simulink model "WarehousePhase2Sim"  (R2024b)
settings: Solver=ode4  StartTime=0.0  StopTime=inf  FixedStep=0.02  RelTol=1e-3
StopFcn:
  | try, fleetVisionStep('close'); catch, end; try, phase2('stopped'); catch, end
model workspace (MAT data in the model file):
  HomePose1 = [-20 7.3 0]
  Zero = 0
  gen3 : robotics.RigidBodyTree (value not decoded)
  qStow = [0; 0; 0.261799387799; 3.14159265359; -2.26892802759; 0; 0.959931088597; 1.57079632679]
undefined symbols (not defined in the file or in its folder): Actor, setupFleetScene, Sim3dSensor, World
libraries: sim3dlib x113, sim3dcameralib x2, robotmobilelib x1, robotsim3dlib x1
(part 2 of 2)

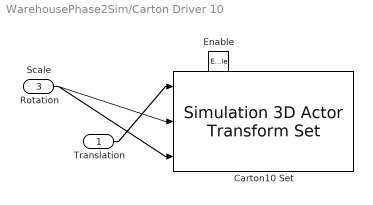
== system WarehousePhase2Sim/Carton Driver 10 ==
  Translation : Inport
  Rotation : Inport  Port=2
  Scale : Inport  Port=3
  Enable : EnablePort
  Carton10 Set : sim3dlib/Simulation 3D Actor Transform Set  Priority=1  ActorTag=Carton10  NumberOfParts=1  CustNumOfParts=3  Translation=[0 0 0]  Rotation=[0 0 0]  Scale=[1 1 1]  Ts=-1  aMode=aMode
  wires:
  Translation/1 -> Carton10 Set/1
  Rotation/1 -> Carton10 Set/2
  Scale/1 -> Carton10 Set/3

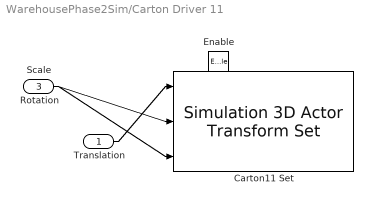
== system WarehousePhase2Sim/Carton Driver 11 ==
  Translation : Inport
  Rotation : Inport  Port=2
  Scale : Inport  Port=3
  Enable : EnablePort
  Carton11 Set : sim3dlib/Simulation 3D Actor Transform Set  Priority=1  ActorTag=Carton11  NumberOfParts=1  CustNumOfParts=3  Translation=[0 0 0]  Rotation=[0 0 0]  Scale=[1 1 1]  Ts=-1  aMode=aMode
  wires:
  Translation/1 -> Carton11 Set/1
  Rotation/1 -> Carton11 Set/2
  Scale/1 -> Carton11 Set/3

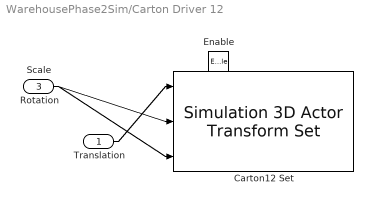
== system WarehousePhase2Sim/Carton Driver 12 ==
  Translation : Inport
  Rotation : Inport  Port=2
  Scale : Inport  Port=3
  Enable : EnablePort
  Carton12 Set : sim3dlib/Simulation 3D Actor Transform Set  Priority=1  ActorTag=Carton12  NumberOfParts=1  CustNumOfParts=3  Translation=[0 0 0]  Rotation=[0 0 0]  Scale=[1 1 1]  Ts=-1  aMode=aMode
  wires:
  Translation/1 -> Carton12 Set/1
  Rotation/1 -> Carton12 Set/2
  Scale/1 -> Carton12 Set/3

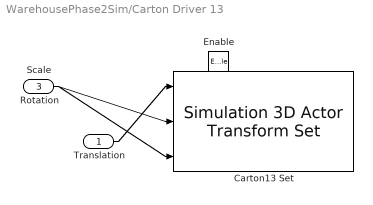
== system WarehousePhase2Sim/Carton Driver 13 ==
  Translation : Inport
  Rotation : Inport  Port=2
  Scale : Inport  Port=3
  Enable : EnablePort
  Carton13 Set : sim3dlib/Simulation 3D Actor Transform Set  Priority=1  ActorTag=Carton13  NumberOfParts=1  CustNumOfParts=3  Translation=[0 0 0]  Rotation=[0 0 0]  Scale=[1 1 1]  Ts=-1  aMode=aMode
  wires:
  Translation/1 -> Carton13 Set/1
  Rotation/1 -> Carton13 Set/2
  Scale/1 -> Carton13 Set/3

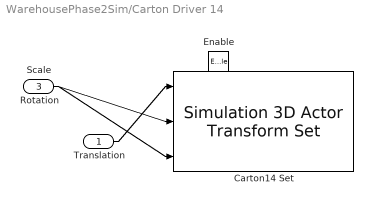
== system WarehousePhase2Sim/Carton Driver 14 ==
  Translation : Inport
  Rotation : Inport  Port=2
  Scale : Inport  Port=3
  Enable : EnablePort
  Carton14 Set : sim3dlib/Simulation 3D Actor Transform Set  Priority=1  ActorTag=Carton14  NumberOfParts=1  CustNumOfParts=3  Translation=[0 0 0]  Rotation=[0 0 0]  Scale=[1 1 1]  Ts=-1  aMode=aMode
  wires:
  Translation/1 -> Carton14 Set/1
  Rotation/1 -> Carton14 Set/2
  Scale/1 -> Carton14 Set/3

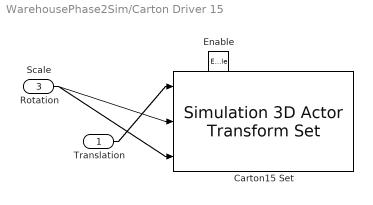
== system WarehousePhase2Sim/Carton Driver 15 ==
  Translation : Inport
  Rotation : Inport  Port=2
  Scale : Inport  Port=3
  Enable : EnablePort
  Carton15 Set : sim3dlib/Simulation 3D Actor Transform Set  Priority=1  ActorTag=Carton15  NumberOfParts=1  CustNumOfParts=3  Translation=[0 0 0]  Rotation=[0 0 0]  Scale=[1 1 1]  Ts=-1  aMode=aMode
  wires:
  Translation/1 -> Carton15 Set/1
  Rotation/1 -> Carton15 Set/2
  Scale/1 -> Carton15 Set/3

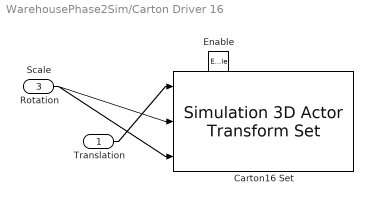
== system WarehousePhase2Sim/Carton Driver 16 ==
  Translation : Inport
  Rotation : Inport  Port=2
  Scale : Inport  Port=3
  Enable : EnablePort
  Carton16 Set : sim3dlib/Simulation 3D Actor Transform Set  Priority=1  ActorTag=Carton16  NumberOfParts=1  CustNumOfParts=3  Translation=[0 0 0]  Rotation=[0 0 0]  Scale=[1 1 1]  Ts=-1  aMode=aMode
  wires:
  Translation/1 -> Carton16 Set/1
  Rotation/1 -> Carton16 Set/2
  Scale/1 -> Carton16 Set/3

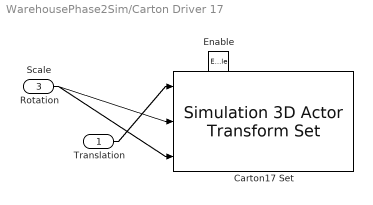
== system WarehousePhase2Sim/Carton Driver 17 ==
  Translation : Inport
  Rotation : Inport  Port=2
  Scale : Inport  Port=3
  Enable : EnablePort
  Carton17 Set : sim3dlib/Simulation 3D Actor Transform Set  Priority=1  ActorTag=Carton17  NumberOfParts=1  CustNumOfParts=3  Translation=[0 0 0]  Rotation=[0 0 0]  Scale=[1 1 1]  Ts=-1  aMode=aMode
  wires:
  Translation/1 -> Carton17 Set/1
  Rotation/1 -> Carton17 Set/2
  Scale/1 -> Carton17 Set/3

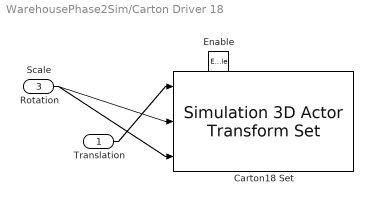
== system WarehousePhase2Sim/Carton Driver 18 ==
  Translation : Inport
  Rotation : Inport  Port=2
  Scale : Inport  Port=3
  Enable : EnablePort
  Carton18 Set : sim3dlib/Simulation 3D Actor Transform Set  Priority=1  ActorTag=Carton18  NumberOfParts=1  CustNumOfParts=3  Translation=[0 0 0]  Rotation=[0 0 0]  Scale=[1 1 1]  Ts=-1  aMode=aMode
  wires:
  Translation/1 -> Carton18 Set/1
  Rotation/1 -> Carton18 Set/2
  Scale/1 -> Carton18 Set/3

== system WarehousePhase2Sim/Carton Driver 19 ==
  Translation : Inport
  Rotation : Inport  Port=2
  Scale : Inport  Port=3
  Enable : EnablePort
  Carton19 Set : sim3dlib/Simulation 3D Actor Transform Set  Priority=1  ActorTag=Carton19  NumberOfParts=1  CustNumOfParts=3  Translation=[0 0 0]  Rotation=[0 0 0]  Scale=[1 1 1]  Ts=-1  aMode=aMode
  wires:
  Translation/1 -> Carton19 Set/1
  Rotation/1 -> Carton19 Set/2
  Scale/1 -> Carton19 Set/3

== system WarehousePhase2Sim/Carton Driver 2 ==
  Translation : Inport
  Rotation : Inport  Port=2
  Scale : Inport  Port=3
  Enable : EnablePort
  Carton02 Set : sim3dlib/Simulation 3D Actor Transform Set  Priority=1  ActorTag=Carton02  NumberOfParts=1  CustNumOfParts=3  Translation=[0 0 0]  Rotation=[0 0 0]  Scale=[1 1 1]  Ts=-1  aMode=aMode
  wires:
  Translation/1 -> Carton02 Set/1
  Rotation/1 -> Carton02 Set/2
  Scale/1 -> Carton02 Set/3

== system WarehousePhase2Sim/Carton Driver 20 ==
  Translation : Inport
  Rotation : Inport  Port=2
  Scale : Inport  Port=3
  Enable : EnablePort
  Carton20 Set : sim3dlib/Simulation 3D Actor Transform Set  Priority=1  ActorTag=Carton20  NumberOfParts=1  CustNumOfParts=3  Translation=[0 0 0]  Rotation=[0 0 0]  Scale=[1 1 1]  Ts=-1  aMode=aMode
  wires:
  Translation/1 -> Carton20 Set/1
  Rotation/1 -> Carton20 Set/2
  Scale/1 -> Carton20 Set/3

== system WarehousePhase2Sim/Carton Driver 21 ==
  Translation : Inport
  Rotation : Inport  Port=2
  Scale : Inport  Port=3
  Enable : EnablePort
  Carton21 Set : sim3dlib/Simulation 3D Actor Transform Set  Priority=1  ActorTag=Carton21  NumberOfParts=1  CustNumOfParts=3  Translation=[0 0 0]  Rotation=[0 0 0]  Scale=[1 1 1]  Ts=-1  aMode=aMode
  wires:
  Translation/1 -> Carton21 Set/1
  Rotation/1 -> Carton21 Set/2
  Scale/1 -> Carton21 Set/3

== system WarehousePhase2Sim/Carton Driver 22 ==
  Translation : Inport
  Rotation : Inport  Port=2
  Scale : Inport  Port=3
  Enable : EnablePort
  Carton22 Set : sim3dlib/Simulation 3D Actor Transform Set  Priority=1  ActorTag=Carton22  NumberOfParts=1  CustNumOfParts=3  Translation=[0 0 0]  Rotation=[0 0 0]  Scale=[1 1 1]  Ts=-1  aMode=aMode
  wires:
  Translation/1 -> Carton22 Set/1
  Rotation/1 -> Carton22 Set/2
  Scale/1 -> Carton22 Set/3

== system WarehousePhase2Sim/Carton Driver 23 ==
  Translation : Inport
  Rotation : Inport  Port=2
  Scale : Inport  Port=3
  Enable : EnablePort
  Carton23 Set : sim3dlib/Simulation 3D Actor Transform Set  Priority=1  ActorTag=Carton23  NumberOfParts=1  CustNumOfParts=3  Translation=[0 0 0]  Rotation=[0 0 0]  Scale=[1 1 1]  Ts=-1  aMode=aMode
  wires:
  Translation/1 -> Carton23 Set/1
  Rotation/1 -> Carton23 Set/2
  Scale/1 -> Carton23 Set/3

== system WarehousePhase2Sim/Carton Driver 24 ==
  Translation : Inport
  Rotation : Inport  Port=2
  Scale : Inport  Port=3
  Enable : EnablePort
  Carton24 Set : sim3dlib/Simulation 3D Actor Transform Set  Priority=1  ActorTag=Carton24  NumberOfParts=1  CustNumOfParts=3  Translation=[0 0 0]  Rotation=[0 0 0]  Scale=[1 1 1]  Ts=-1  aMode=aMode
  wires:
  Translation/1 -> Carton24 Set/1
  Rotation/1 -> Carton24 Set/2
  Scale/1 -> Carton24 Set/3

== system WarehousePhase2Sim/Carton Driver 25 ==
  Translation : Inport
  Rotation : Inport  Port=2
  Scale : Inport  Port=3
  Enable : EnablePort
  Carton25 Set : sim3dlib/Simulation 3D Actor Transform Set  Priority=1  ActorTag=Carton25  NumberOfParts=1  CustNumOfParts=3  Translation=[0 0 0]  Rotation=[0 0 0]  Scale=[1 1 1]  Ts=-1  aMode=aMode
  wires:
  Translation/1 -> Carton25 Set/1
  Rotation/1 -> Carton25 Set/2
  Scale/1 -> Carton25 Set/3

== system WarehousePhase2Sim/Carton Driver 26 ==
  Translation : Inport
  Rotation : Inport  Port=2
  Scale : Inport  Port=3
  Enable : EnablePort
  Carton26 Set : sim3dlib/Simulation 3D Actor Transform Set  Priority=1  ActorTag=Carton26  NumberOfParts=1  CustNumOfParts=3  Translation=[0 0 0]  Rotation=[0 0 0]  Scale=[1 1 1]  Ts=-1  aMode=aMode
  wires:
  Translation/1 -> Carton26 Set/1
  Rotation/1 -> Carton26 Set/2
  Scale/1 -> Carton26 Set/3

== system WarehousePhase2Sim/Carton Driver 27 ==
  Translation : Inport
  Rotation : Inport  Port=2
  Scale : Inport  Port=3
  Enable : EnablePort
  Carton27 Set : sim3dlib/Simulation 3D Actor Transform Set  Priority=1  ActorTag=Carton27  NumberOfParts=1  CustNumOfParts=3  Translation=[0 0 0]  Rotation=[0 0 0]  Scale=[1 1 1]  Ts=-1  aMode=aMode
  wires:
  Translation/1 -> Carton27 Set/1
  Rotation/1 -> Carton27 Set/2
  Scale/1 -> Carton27 Set/3

== system WarehousePhase2Sim/Carton Driver 28 ==
  Translation : Inport
  Rotation : Inport  Port=2
  Scale : Inport  Port=3
  Enable : EnablePort
  Carton28 Set : sim3dlib/Simulation 3D Actor Transform Set  Priority=1  ActorTag=Carton28  NumberOfParts=1  CustNumOfParts=3  Translation=[0 0 0]  Rotation=[0 0 0]  Scale=[1 1 1]  Ts=-1  aMode=aMode
  wires:
  Translation/1 -> Carton28 Set/1
  Rotation/1 -> Carton28 Set/2
  Scale/1 -> Carton28 Set/3

== system WarehousePhase2Sim/Carton Driver 29 ==
  Translation : Inport
  Rotation : Inport  Port=2
  Scale : Inport  Port=3
  Enable : EnablePort
  Carton29 Set : sim3dlib/Simulation 3D Actor Transform Set  Priority=1  ActorTag=Carton29  NumberOfParts=1  CustNumOfParts=3  Translation=[0 0 0]  Rotation=[0 0 0]  Scale=[1 1 1]  Ts=-1  aMode=aMode
  wires:
  Translation/1 -> Carton29 Set/1
  Rotation/1 -> Carton29 Set/2
  Scale/1 -> Carton29 Set/3

== system WarehousePhase2Sim/Carton Driver 3 ==
  Translation : Inport
  Rotation : Inport  Port=2
  Scale : Inport  Port=3
  Enable : EnablePort
  Carton03 Set : sim3dlib/Simulation 3D Actor Transform Set  Priority=1  ActorTag=Carton03  NumberOfParts=1  CustNumOfParts=3  Translation=[0 0 0]  Rotation=[0 0 0]  Scale=[1 1 1]  Ts=-1  aMode=aMode
  wires:
  Translation/1 -> Carton03 Set/1
  Rotation/1 -> Carton03 Set/2
  Scale/1 -> Carton03 Set/3

== system WarehousePhase2Sim/Carton Driver 30 ==
  Translation : Inport
  Rotation : Inport  Port=2
  Scale : Inport  Port=3
  Enable : EnablePort
  Carton30 Set : sim3dlib/Simulation 3D Actor Transform Set  Priority=1  ActorTag=Carton30  NumberOfParts=1  CustNumOfParts=3  Translation=[0 0 0]  Rotation=[0 0 0]  Scale=[1 1 1]  Ts=-1  aMode=aMode
  wires:
  Translation/1 -> Carton30 Set/1
  Rotation/1 -> Carton30 Set/2
  Scale/1 -> Carton30 Set/3

== system WarehousePhase2Sim/Carton Driver 31 ==
  Translation : Inport
  Rotation : Inport  Port=2
  Scale : Inport  Port=3
  Enable : EnablePort
  Carton31 Set : sim3dlib/Simulation 3D Actor Transform Set  Priority=1  ActorTag=Carton31  NumberOfParts=1  CustNumOfParts=3  Translation=[0 0 0]  Rotation=[0 0 0]  Scale=[1 1 1]  Ts=-1  aMode=aMode
  wires:
  Translation/1 -> Carton31 Set/1
  Rotation/1 -> Carton31 Set/2
  Scale/1 -> Carton31 Set/3

== system WarehousePhase2Sim/Carton Driver 32 ==
  Translation : Inport
  Rotation : Inport  Port=2
  Scale : Inport  Port=3
  Enable : EnablePort
  Carton32 Set : sim3dlib/Simulation 3D Actor Transform Set  Priority=1  ActorTag=Carton32  NumberOfParts=1  CustNumOfParts=3  Translation=[0 0 0]  Rotation=[0 0 0]  Scale=[1 1 1]  Ts=-1  aMode=aMode
  wires:
  Translation/1 -> Carton32 Set/1
  Rotation/1 -> Carton32 Set/2
  Scale/1 -> Carton32 Set/3

== system WarehousePhase2Sim/Carton Driver 33 ==
  Translation : Inport
  Rotation : Inport  Port=2
  Scale : Inport  Port=3
  Enable : EnablePort
  Carton33 Set : sim3dlib/Simulation 3D Actor Transform Set  Priority=1  ActorTag=Carton33  NumberOfParts=1  CustNumOfParts=3  Translation=[0 0 0]  Rotation=[0 0 0]  Scale=[1 1 1]  Ts=-1  aMode=aMode
  wires:
  Translation/1 -> Carton33 Set/1
  Rotation/1 -> Carton33 Set/2
  Scale/1 -> Carton33 Set/3

== system WarehousePhase2Sim/Carton Driver 34 ==
  Translation : Inport
  Rotation : Inport  Port=2
  Scale : Inport  Port=3
  Enable : EnablePort
  Carton34 Set : sim3dlib/Simulation 3D Actor Transform Set  Priority=1  ActorTag=Carton34  NumberOfParts=1  CustNumOfParts=3  Translation=[0 0 0]  Rotation=[0 0 0]  Scale=[1 1 1]  Ts=-1  aMode=aMode
  wires:
  Translation/1 -> Carton34 Set/1
  Rotation/1 -> Carton34 Set/2
  Scale/1 -> Carton34 Set/3

== system WarehousePhase2Sim/Carton Driver 35 ==
  Translation : Inport
  Rotation : Inport  Port=2
  Scale : Inport  Port=3
  Enable : EnablePort
  Carton35 Set : sim3dlib/Simulation 3D Actor Transform Set  Priority=1  ActorTag=Carton35  NumberOfParts=1  CustNumOfParts=3  Translation=[0 0 0]  Rotation=[0 0 0]  Scale=[1 1 1]  Ts=-1  aMode=aMode
  wires:
  Translation/1 -> Carton35 Set/1
  Rotation/1 -> Carton35 Set/2
  Scale/1 -> Carton35 Set/3

== system WarehousePhase2Sim/Carton Driver 36 ==
  Translation : Inport
  Rotation : Inport  Port=2
  Scale : Inport  Port=3
  Enable : EnablePort
  Carton36 Set : sim3dlib/Simulation 3D Actor Transform Set  Priority=1  ActorTag=Carton36  NumberOfParts=1  CustNumOfParts=3  Translation=[0 0 0]  Rotation=[0 0 0]  Scale=[1 1 1]  Ts=-1  aMode=aMode
  wires:
  Translation/1 -> Carton36 Set/1
  Rotation/1 -> Carton36 Set/2
  Scale/1 -> Carton36 Set/3

== system WarehousePhase2Sim/Carton Driver 37 ==
  Translation : Inport
  Rotation : Inport  Port=2
  Scale : Inport  Port=3
  Enable : EnablePort
  Carton37 Set : sim3dlib/Simulation 3D Actor Transform Set  Priority=1  ActorTag=Carton37  NumberOfParts=1  CustNumOfParts=3  Translation=[0 0 0]  Rotation=[0 0 0]  Scale=[1 1 1]  Ts=-1  aMode=aMode
  wires:
  Translation/1 -> Carton37 Set/1
  Rotation/1 -> Carton37 Set/2
  Scale/1 -> Carton37 Set/3

== system WarehousePhase2Sim/Carton Driver 38 ==
  Translation : Inport
  Rotation : Inport  Port=2
  Scale : Inport  Port=3
  Enable : EnablePort
  Carton38 Set : sim3dlib/Simulation 3D Actor Transform Set  Priority=1  ActorTag=Carton38  NumberOfParts=1  CustNumOfParts=3  Translation=[0 0 0]  Rotation=[0 0 0]  Scale=[1 1 1]  Ts=-1  aMode=aMode
  wires:
  Translation/1 -> Carton38 Set/1
  Rotation/1 -> Carton38 Set/2
  Scale/1 -> Carton38 Set/3

== system WarehousePhase2Sim/Carton Driver 39 ==
  Translation : Inport
  Rotation : Inport  Port=2
  Scale : Inport  Port=3
  Enable : EnablePort
  Carton39 Set : sim3dlib/Simulation 3D Actor Transform Set  Priority=1  ActorTag=Carton39  NumberOfParts=1  CustNumOfParts=3  Translation=[0 0 0]  Rotation=[0 0 0]  Scale=[1 1 1]  Ts=-1  aMode=aMode
  wires:
  Translation/1 -> Carton39 Set/1
  Rotation/1 -> Carton39 Set/2
  Scale/1 -> Carton39 Set/3

== system WarehousePhase2Sim/Carton Driver 4 ==
  Translation : Inport
  Rotation : Inport  Port=2
  Scale : Inport  Port=3
  Enable : EnablePort
  Carton04 Set : sim3dlib/Simulation 3D Actor Transform Set  Priority=1  ActorTag=Carton04  NumberOfParts=1  CustNumOfParts=3  Translation=[0 0 0]  Rotation=[0 0 0]  Scale=[1 1 1]  Ts=-1  aMode=aMode
  wires:
  Translation/1 -> Carton04 Set/1
  Rotation/1 -> Carton04 Set/2
  Scale/1 -> Carton04 Set/3

== system WarehousePhase2Sim/Carton Driver 40 ==
  Translation : Inport
  Rotation : Inport  Port=2
  Scale : Inport  Port=3
  Enable : EnablePort
  Carton40 Set : sim3dlib/Simulation 3D Actor Transform Set  Priority=1  ActorTag=Carton40  NumberOfParts=1  CustNumOfParts=3  Translation=[0 0 0]  Rotation=[0 0 0]  Scale=[1 1 1]  Ts=-1  aMode=aMode
  wires:
  Translation/1 -> Carton40 Set/1
  Rotation/1 -> Carton40 Set/2
  Scale/1 -> Carton40 Set/3

== system WarehousePhase2Sim/Carton Driver 41 ==
  Translation : Inport
  Rotation : Inport  Port=2
  Scale : Inport  Port=3
  Enable : EnablePort
  Carton41 Set : sim3dlib/Simulation 3D Actor Transform Set  Priority=1  ActorTag=Carton41  NumberOfParts=1  CustNumOfParts=3  Translation=[0 0 0]  Rotation=[0 0 0]  Scale=[1 1 1]  Ts=-1  aMode=aMode
  wires:
  Translation/1 -> Carton41 Set/1
  Rotation/1 -> Carton41 Set/2
  Scale/1 -> Carton41 Set/3

== system WarehousePhase2Sim/Carton Driver 42 ==
  Translation : Inport
  Rotation : Inport  Port=2
  Scale : Inport  Port=3
  Enable : EnablePort
  Carton42 Set : sim3dlib/Simulation 3D Actor Transform Set  Priority=1  ActorTag=Carton42  NumberOfParts=1  CustNumOfParts=3  Translation=[0 0 0]  Rotation=[0 0 0]  Scale=[1 1 1]  Ts=-1  aMode=aMode
  wires:
  Translation/1 -> Carton42 Set/1
  Rotation/1 -> Carton42 Set/2
  Scale/1 -> Carton42 Set/3

== system WarehousePhase2Sim/Carton Driver 43 ==
  Translation : Inport
  Rotation : Inport  Port=2
  Scale : Inport  Port=3
  Enable : EnablePort
  Carton43 Set : sim3dlib/Simulation 3D Actor Transform Set  Priority=1  ActorTag=Carton43  NumberOfParts=1  CustNumOfParts=3  Translation=[0 0 0]  Rotation=[0 0 0]  Scale=[1 1 1]  Ts=-1  aMode=aMode
  wires:
  Translation/1 -> Carton43 Set/1
  Rotation/1 -> Carton43 Set/2
  Scale/1 -> Carton43 Set/3

== system WarehousePhase2Sim/Carton Driver 44 ==
  Translation : Inport
  Rotation : Inport  Port=2
  Scale : Inport  Port=3
  Enable : EnablePort
  Carton44 Set : sim3dlib/Simulation 3D Actor Transform Set  Priority=1  ActorTag=Carton44  NumberOfParts=1  CustNumOfParts=3  Translation=[0 0 0]  Rotation=[0 0 0]  Scale=[1 1 1]  Ts=-1  aMode=aMode
  wires:
  Translation/1 -> Carton44 Set/1
  Rotation/1 -> Carton44 Set/2
  Scale/1 -> Carton44 Set/3

== system WarehousePhase2Sim/Carton Driver 45 ==
  Translation : Inport
  Rotation : Inport  Port=2
  Scale : Inport  Port=3
  Enable : EnablePort
  Carton45 Set : sim3dlib/Simulation 3D Actor Transform Set  Priority=1  ActorTag=Carton45  NumberOfParts=1  CustNumOfParts=3  Translation=[0 0 0]  Rotation=[0 0 0]  Scale=[1 1 1]  Ts=-1  aMode=aMode
  wires:
  Translation/1 -> Carton45 Set/1
  Rotation/1 -> Carton45 Set/2
  Scale/1 -> Carton45 Set/3

== system WarehousePhase2Sim/Carton Driver 46 ==
  Translation : Inport
  Rotation : Inport  Port=2
  Scale : Inport  Port=3
  Enable : EnablePort
  Carton46 Set : sim3dlib/Simulation 3D Actor Transform Set  Priority=1  ActorTag=Carton46  NumberOfParts=1  CustNumOfParts=3  Translation=[0 0 0]  Rotation=[0 0 0]  Scale=[1 1 1]  Ts=-1  aMode=aMode
  wires:
  Translation/1 -> Carton46 Set/1
  Rotation/1 -> Carton46 Set/2
  Scale/1 -> Carton46 Set/3

== system WarehousePhase2Sim/Carton Driver 47 ==
  Translation : Inport
  Rotation : Inport  Port=2
  Scale : Inport  Port=3
  Enable : EnablePort
  Carton47 Set : sim3dlib/Simulation 3D Actor Transform Set  Priority=1  ActorTag=Carton47  NumberOfParts=1  CustNumOfParts=3  Translation=[0 0 0]  Rotation=[0 0 0]  Scale=[1 1 1]  Ts=-1  aMode=aMode
  wires:
  Translation/1 -> Carton47 Set/1
  Rotation/1 -> Carton47 Set/2
  Scale/1 -> Carton47 Set/3

== system WarehousePhase2Sim/Carton Driver 48 ==
  Translation : Inport
  Rotation : Inport  Port=2
  Scale : Inport  Port=3
  Enable : EnablePort
  Carton48 Set : sim3dlib/Simulation 3D Actor Transform Set  Priority=1  ActorTag=Carton48  NumberOfParts=1  CustNumOfParts=3  Translation=[0 0 0]  Rotation=[0 0 0]  Scale=[1 1 1]  Ts=-1  aMode=aMode
  wires:
  Translation/1 -> Carton48 Set/1
  Rotation/1 -> Carton48 Set/2
  Scale/1 -> Carton48 Set/3

== system WarehousePhase2Sim/Carton Driver 49 ==
  Translation : Inport
  Rotation : Inport  Port=2
  Scale : Inport  Port=3
  Enable : EnablePort
  Carton49 Set : sim3dlib/Simulation 3D Actor Transform Set  Priority=1  ActorTag=Carton49  NumberOfParts=1  CustNumOfParts=3  Translation=[0 0 0]  Rotation=[0 0 0]  Scale=[1 1 1]  Ts=-1  aMode=aMode
  wires:
  Translation/1 -> Carton49 Set/1
  Rotation/1 -> Carton49 Set/2
  Scale/1 -> Carton49 Set/3

== system WarehousePhase2Sim/Carton Driver 5 ==
  Translation : Inport
  Rotation : Inport  Port=2
  Scale : Inport  Port=3
  Enable : EnablePort
  Carton05 Set : sim3dlib/Simulation 3D Actor Transform Set  Priority=1  ActorTag=Carton05  NumberOfParts=1  CustNumOfParts=3  Translation=[0 0 0]  Rotation=[0 0 0]  Scale=[1 1 1]  Ts=-1  aMode=aMode
  wires:
  Translation/1 -> Carton05 Set/1
  Rotation/1 -> Carton05 Set/2
  Scale/1 -> Carton05 Set/3

== system WarehousePhase2Sim/Carton Driver 50 ==
  Translation : Inport
  Rotation : Inport  Port=2
  Scale : Inport  Port=3
  Enable : EnablePort
  Carton50 Set : sim3dlib/Simulation 3D Actor Transform Set  Priority=1  ActorTag=Carton50  NumberOfParts=1  CustNumOfParts=3  Translation=[0 0 0]  Rotation=[0 0 0]  Scale=[1 1 1]  Ts=-1  aMode=aMode
  wires:
  Translation/1 -> Carton50 Set/1
  Rotation/1 -> Carton50 Set/2
  Scale/1 -> Carton50 Set/3

== system WarehousePhase2Sim/Carton Driver 51 ==
  Translation : Inport
  Rotation : Inport  Port=2
  Scale : Inport  Port=3
  Enable : EnablePort
  Carton51 Set : sim3dlib/Simulation 3D Actor Transform Set  Priority=1  ActorTag=Carton51  NumberOfParts=1  CustNumOfParts=3  Translation=[0 0 0]  Rotation=[0 0 0]  Scale=[1 1 1]  Ts=-1  aMode=aMode
  wires:
  Translation/1 -> Carton51 Set/1
  Rotation/1 -> Carton51 Set/2
  Scale/1 -> Carton51 Set/3

== system WarehousePhase2Sim/Carton Driver 52 ==
  Translation : Inport
  Rotation : Inport  Port=2
  Scale : Inport  Port=3
  Enable : EnablePort
  Carton52 Set : sim3dlib/Simulation 3D Actor Transform Set  Priority=1  ActorTag=Carton52  NumberOfParts=1  CustNumOfParts=3  Translation=[0 0 0]  Rotation=[0 0 0]  Scale=[1 1 1]  Ts=-1  aMode=aMode
  wires:
  Translation/1 -> Carton52 Set/1
  Rotation/1 -> Carton52 Set/2
  Scale/1 -> Carton52 Set/3

== system WarehousePhase2Sim/Carton Driver 53 ==
  Translation : Inport
  Rotation : Inport  Port=2
  Scale : Inport  Port=3
  Enable : EnablePort
  Carton53 Set : sim3dlib/Simulation 3D Actor Transform Set  Priority=1  ActorTag=Carton53  NumberOfParts=1  CustNumOfParts=3  Translation=[0 0 0]  Rotation=[0 0 0]  Scale=[1 1 1]  Ts=-1  aMode=aMode
  wires:
  Translation/1 -> Carton53 Set/1
  Rotation/1 -> Carton53 Set/2
  Scale/1 -> Carton53 Set/3

== system WarehousePhase2Sim/Carton Driver 54 ==
  Translation : Inport
  Rotation : Inport  Port=2
  Scale : Inport  Port=3
  Enable : EnablePort
  Carton54 Set : sim3dlib/Simulation 3D Actor Transform Set  Priority=1  ActorTag=Carton54  NumberOfParts=1  CustNumOfParts=3  Translation=[0 0 0]  Rotation=[0 0 0]  Scale=[1 1 1]  Ts=-1  aMode=aMode
  wires:
  Translation/1 -> Carton54 Set/1
  Rotation/1 -> Carton54 Set/2
  Scale/1 -> Carton54 Set/3

== system WarehousePhase2Sim/Carton Driver 6 ==
  Translation : Inport
  Rotation : Inport  Port=2
  Scale : Inport  Port=3
  Enable : EnablePort
  Carton06 Set : sim3dlib/Simulation 3D Actor Transform Set  Priority=1  ActorTag=Carton06  NumberOfParts=1  CustNumOfParts=3  Translation=[0 0 0]  Rotation=[0 0 0]  Scale=[1 1 1]  Ts=-1  aMode=aMode
  wires:
  Translation/1 -> Carton06 Set/1
  Rotation/1 -> Carton06 Set/2
  Scale/1 -> Carton06 Set/3

== system WarehousePhase2Sim/Carton Driver 7 ==
  Translation : Inport
  Rotation : Inport  Port=2
  Scale : Inport  Port=3
  Enable : EnablePort
  Carton07 Set : sim3dlib/Simulation 3D Actor Transform Set  Priority=1  ActorTag=Carton07  NumberOfParts=1  CustNumOfParts=3  Translation=[0 0 0]  Rotation=[0 0 0]  Scale=[1 1 1]  Ts=-1  aMode=aMode
  wires:
  Translation/1 -> Carton07 Set/1
  Rotation/1 -> Carton07 Set/2
  Scale/1 -> Carton07 Set/3

== system WarehousePhase2Sim/Carton Driver 8 ==
  Translation : Inport
  Rotation : Inport  Port=2
  Scale : Inport  Port=3
  Enable : EnablePort
  Carton08 Set : sim3dlib/Simulation 3D Actor Transform Set  Priority=1  ActorTag=Carton08  NumberOfParts=1  CustNumOfParts=3  Translation=[0 0 0]  Rotation=[0 0 0]  Scale=[1 1 1]  Ts=-1  aMode=aMode
  wires:
  Translation/1 -> Carton08 Set/1
  Rotation/1 -> Carton08 Set/2
  Scale/1 -> Carton08 Set/3

== system WarehousePhase2Sim/Carton Driver 9 ==
  Translation : Inport
  Rotation : Inport  Port=2
  Scale : Inport  Port=3
  Enable : EnablePort
  Carton09 Set : sim3dlib/Simulation 3D Actor Transform Set  Priority=1  ActorTag=Carton09  NumberOfParts=1  CustNumOfParts=3  Translation=[0 0 0]  Rotation=[0 0 0]  Scale=[1 1 1]  Ts=-1  aMode=aMode
  wires:
  Translation/1 -> Carton09 Set/1
  Rotation/1 -> Carton09 Set/2
  Scale/1 -> Carton09 Set/3

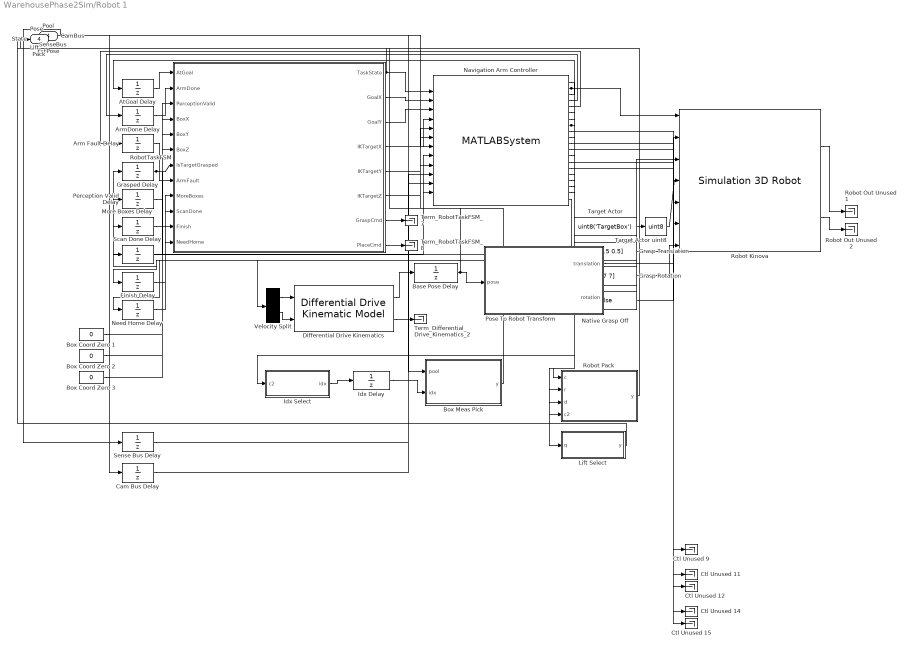
== system WarehousePhase2Sim/Robot 1 ==
  Pool : Inport
  EstPose : Inport  Port=2
  SenseBus : Inport  Port=3
  CamBus : Inport  Port=4
  Arm Fault Delay : UnitDelay  InitialCondition=false  SampleTime=0.02  HasFrameUpgradeWarning=on
  ArmDone Delay : UnitDelay  InitialCondition=false  SampleTime=0.02  HasFrameUpgradeWarning=on
  AtGoal Delay : UnitDelay  InitialCondition=false  SampleTime=0.02  HasFrameUpgradeWarning=on
  Base Pose Delay : UnitDelay  InitialCondition=HomePose1  SampleTime=0.02  HasFrameUpgradeWarning=on
  Box Coord Zero 1 : Constant  Value=0  OutDataTypeStr=double
  Box Coord Zero 2 : Constant  Value=0  OutDataTypeStr=double
  Box Coord Zero 3 : Constant  Value=0  OutDataTypeStr=double
  Box Meas Pick : MATLAB Function  TreatAsAtomicUnit=on
  Cam Bus Delay : UnitDelay  InitialCondition=zeros(1,8)  SampleTime=0.02  HasFrameUpgradeWarning=on
  Ctl Unused {9,11..12,14..15} (5 alike) : Terminator
  Differential Drive Kinematics : robotmobilelib/Differential Drive Kinematic Model  VehicleInputs=Vehicle Speed & Heading Angular Velocity  WheelRadius=0.05  WheelSpeedRange=[-inf inf]  TrackWidth=0.2  InitialState=HomePose1  SimulateUsing=Interpreted execution
  Finish Delay : UnitDelay  InitialCondition=false  SampleTime=0.02  HasFrameUpgradeWarning=on
  Grasp Rotation : Constant  Value=[7 7 7]
  Grasp Translation : Constant  Value=[0.5 0.5 0.5]
  Grasped Delay : UnitDelay  InitialCondition=false  SampleTime=0.02  HasFrameUpgradeWarning=on
  Idx Delay : UnitDelay  SampleTime=0.02  HasFrameUpgradeWarning=on
  Idx Select : MATLAB Function  TreatAsAtomicUnit=on
  Lift Select : MATLAB Function  TreatAsAtomicUnit=on
  More Boxes Delay : UnitDelay  InitialCondition=false  SampleTime=0.02  HasFrameUpgradeWarning=on
  Native Grasp Off : Constant  Value=false  OutDataTypeStr=boolean
  Navigation Arm Controller : MATLABSystem  System=WarehouseRobotControlSystemV23  SampleTime=0.02  RobotId=1  SimulateUsing=Interpreted execution
      mask Type: WarehouseRobotControlSystemV23
      mask Display:
      | disp('WarehouseRobotControlSystemV23');
      | port_label('input',1,'state');
      | port_label('input',2,'~');
      | port_label('input',3,'~');
      | port_label('input',4,'~');
      | port_label('input',5,'~');
      | port_label('input',6,'~');
      | port_label('input',7,'basePose');
      | port_label('input',8,'isTargetGrasped');
      | port_label('input',9,'boxMeas');
      | port_label('input',10,'senseBus');
      | port_label('input',11,'camBus');
      | port_label('input',12,'truePose');
      | port_label('output',1,'velocity');
      | port_label('output',2,'config');
      | port_label('output',3,'atGoal');
      | port_label('output',4,'armDone');
      | port_label('output',5,'armFault');
      | port_label('output',6,'vacuum');
      | port_label('output',7,'c1');
      | port_label('output',8,'c2');
      | port_label('output',9,'c3');
      | port_label('output',10,'r1');
      | port_label('output',11,'r2');
      | port_label('output',12,'r3');
      | port_label('output',13,'d1');
      | port_label('output',14,'d2');
      | port_label('output',15,'d3');
      | port_label('output',16,'percValid');
      | port_label('output',17,'moreBoxes');
      | port_label('output',18,'scanDone');
      | port_label('output',19,'finish');
      | port_label('output',20,'needHome');
  Need Home Delay : UnitDelay  InitialCondition=false  SampleTime=0.02  HasFrameUpgradeWarning=on
  Perception Valid Delay : UnitDelay  InitialCondition=false  SampleTime=0.02  HasFrameUpgradeWarning=on
  Pose To Robot Transform : MATLAB Function  TreatAsAtomicUnit=on
  Robot Kinova : robotsim3dlib/Simulation 3D Robot  Priority=2  actorInputType=RigidBodyTree Object  RigidBodyTree=gen3  ActorName=Ro1Kinova  existActorChekBox=off  initialTrans=[0 0 0]  initialRot=[0 0 0]  initialConfig=qStow  EndEffector=ToolTip  eeOffsetInpChekBox=off  eeTargetTrans=[-0.04 0 0.245]  eeTargetRot=[0 1.2217 3.1416]  enableRegionGraspChekBox=on  regionGraspInpChekBox=on  eeTargTransDiff=[0.2 0.2 0.2]  eeTargRotDiff=[0 0 0]  inpConfEnbVal=on  inpGraspEnbVal=on  inpTransEnbVal=on  outConfEnbVal=on  outGraspEnbVal=on  outTransEnbVal=off  SampleTime=0.02  ActorType=SimulinkVehicle  ID=C  aMode=6  ActorTag=Ro1Kinova  Mesh=RigidBodyTree
  Robot Out Unused 1 : Terminator
  Robot Out Unused 2 : Terminator
  Robot Pack : MATLAB Function  TreatAsAtomicUnit=on
  RobotTaskFSM : Stateflow chart  TreatAsAtomicUnit=on
  Scan Done Delay : UnitDelay  InitialCondition=false  SampleTime=0.02  HasFrameUpgradeWarning=on
  Sense Bus Delay : UnitDelay  InitialCondition=zeros(1,8)  SampleTime=0.02  HasFrameUpgradeWarning=on
  Target Actor : Constant  Value=uint8('TargetBox')  OutDataTypeStr=uint8
  Target Actor uint8 : DataTypeConversion  OutDataTypeStr=uint8  SaturateOnIntegerOverflow=off  RndMeth=Floor
  Term_Differential_Drive_Kinematics_2 : Terminator
  Term_RobotTaskFSM_7 : Terminator
  Term_RobotTaskFSM_8 : Terminator
  Velocity Split : Demux  Outputs=2
  Pose : Outport
  Pack : Outport  Port=2
  Lift : Outport  Port=3
  State : Outport  Port=4
  wires:
  Navigation Arm Controller/3 -> AtGoal Delay/1
  AtGoal Delay/1 -> RobotTaskFSM/1(AtGoal)
  Navigation Arm Controller/4 -> ArmDone Delay/1
  ArmDone Delay/1 -> RobotTaskFSM/2(ArmDone)
  Navigation Arm Controller/5 -> Arm Fault Delay/1
  Arm Fault Delay/1 -> RobotTaskFSM/8(ArmFault)
  Navigation Arm Controller/6 -> Grasped Delay/1
  Grasped Delay/1 -> RobotTaskFSM/7(IsTargetGrasped), Navigation Arm Controller/8
  Navigation Arm Controller/16 -> Perception Valid Delay/1
  Perception Valid Delay/1 -> RobotTaskFSM/3(PerceptionValid)
  Navigation Arm Controller/17 -> More Boxes Delay/1
  More Boxes Delay/1 -> RobotTaskFSM/9(MoreBoxes)
  Navigation Arm Controller/18 -> Scan Done Delay/1
  Scan Done Delay/1 -> RobotTaskFSM/10(ScanDone)
  Navigation Arm Controller/19 -> Finish Delay/1
  Finish Delay/1 -> RobotTaskFSM/11(Finish)
  Navigation Arm Controller/20 -> Need Home Delay/1
  Need Home Delay/1 -> RobotTaskFSM/12(NeedHome)
  Box Coord Zero 1/1 -> RobotTaskFSM/4(BoxX)
  Box Coord Zero 2/1 -> RobotTaskFSM/5(BoxY)
  Box Coord Zero 3/1 -> RobotTaskFSM/6(BoxZ)
  RobotTaskFSM/1(TaskState) -> Navigation Arm Controller/1, State/1
  RobotTaskFSM/2(GoalX) -> Navigation Arm Controller/2
  RobotTaskFSM/3(GoalY) -> Navigation Arm Controller/3
  RobotTaskFSM/4(IKTargetX) -> Navigation Arm Controller/4
  RobotTaskFSM/5(IKTargetY) -> Navigation Arm Controller/5
  RobotTaskFSM/6(IKTargetZ) -> Navigation Arm Controller/6
  EstPose/1 -> Navigation Arm Controller/7
  SenseBus/1 -> Sense Bus Delay/1
  Sense Bus Delay/1 -> Navigation Arm Controller/10
  CamBus/1 -> Cam Bus Delay/1
  Cam Bus Delay/1 -> Navigation Arm Controller/11
  Base Pose Delay/1 -> Navigation Arm Controller/12, Pose/1, Pose To Robot Transform/1(pose)
  Navigation Arm Controller/8 -> Idx Select/1(c2), Robot Pack/4(c2)
  Idx Select/1(idx) -> Idx Delay/1
  Idx Delay/1 -> Box Meas Pick/2(idx)
  Pool/1 -> Box Meas Pick/1(pool)
  Box Meas Pick/1(y) -> Navigation Arm Controller/9
  Navigation Arm Controller/7 -> Robot Pack/1(c)
  Navigation Arm Controller/10 -> Robot Pack/2(r)
  Navigation Arm Controller/13 -> Robot Pack/3(d)
  Robot Pack/1(y) -> Pack/1
  Navigation Arm Controller/2 -> Lift Select/1(q), Robot Kinova/1
  Lift Select/1(y) -> Lift/1
  Navigation Arm Controller/9 -> Ctl Unused 9/1
  Navigation Arm Controller/11 -> Ctl Unused 11/1
  Navigation Arm Controller/12 -> Ctl Unused 12/1
  Navigation Arm Controller/14 -> Ctl Unused 14/1
  Navigation Arm Controller/15 -> Ctl Unused 15/1
  Navigation Arm Controller/1 -> Velocity Split/1
  Velocity Split/1 -> Differential Drive Kinematics/1
  Velocity Split/2 -> Differential Drive Kinematics/2
  Differential Drive Kinematics/1 -> Base Pose Delay/1
  Target Actor/1 -> Target Actor uint8/1
  Pose To Robot Transform/1(translation) -> Robot Kinova/2
  Pose To Robot Transform/2(rotation) -> Robot Kinova/3
  Target Actor uint8/1 -> Robot Kinova/4
  Native Grasp Off/1 -> Robot Kinova/5
  Grasp Translation/1 -> Robot Kinova/6
  Grasp Rotation/1 -> Robot Kinova/7
  Robot Kinova/1 -> Robot Out Unused 1/1
  Robot Kinova/2 -> Robot Out Unused 2/1
  Differential Drive Kinematics/2 -> Term_Differential_Drive_Kinematics_2/1
  RobotTaskFSM/7(GraspCmd) -> Term_RobotTaskFSM_7/1
  RobotTaskFSM/8(PlaceCmd) -> Term_RobotTaskFSM_8/1

== stateflow chart WarehousePhase2Sim/Robot 1/RobotTaskFSM ==
  settings: updateMethod=DISCRETE  sampleTime=0.02
  state IDLE
    en: TaskState=uint8(0); GoalX=-20.0000; GoalY=7.3000; GraspCmd=false; PlaceCmd=false;
  state NAV_TO_STAGING
    en: TaskState=uint8(1); GoalX=15.5000; GoalY=46.0556; GraspCmd=false; PlaceCmd=false;
  state DOCK_SHELF
    en: TaskState=uint8(10); GoalX=14.1900; GoalY=46.0556; IKTargetX=BoxX; IKTargetY=BoxY; IKTargetZ=BoxZ; GraspCmd=false; PlaceCmd=false;
  state ARM_EXTEND
    en: TaskState=uint8(2); IKTargetX=BoxX; IKTargetY=BoxY; IKTargetZ=BoxZ; GraspCmd=false;
  state GRASP
    en: TaskState=uint8(3); GraspCmd=true; PlaceCmd=false;
  state ARM_RETRACT
    en: TaskState=uint8(4); GraspCmd=true; PlaceCmd=false;
  state NAV_TO_TABLE
    en: TaskState=uint8(5); GoalX=18.5000; GoalY=65.1000; GraspCmd=true;
  state ARM_PLACE
    en: TaskState=uint8(6); IKTargetX=18.5000; IKTargetY=65.9700; IKTargetZ=1.0700; GraspCmd=true;
  state RELEASE
    en: TaskState=uint8(8); GraspCmd=false; PlaceCmd=true;
  state ARM_STOW
    en: TaskState=uint8(9); GraspCmd=false; PlaceCmd=false;
  state RETURN_HOME
    en: TaskState=uint8(7); GoalX=-20.0000; GoalY=7.3000; GraspCmd=false;
  state FAULT_HOLD
    en: TaskState=uint8(11); GraspCmd=false; PlaceCmd=false;
  state MISSION_DONE
    en: TaskState=uint8(12); GoalX=-20.0000; GoalY=7.3000; GraspCmd=false; PlaceCmd=false;
  NAV_TO_STAGING -> IDLE [order 2] : [AtGoal && ScanDone && ~PerceptionValid]
  RETURN_HOME -> IDLE : [AtGoal || MoreBoxes]
  (default) -> IDLE
  GRASP -> ARM_RETRACT [order 2] : [ArmDone && IsTargetGrasped]
  DOCK_SHELF -> FAULT_HOLD [order 2] : [ArmFault]
  ARM_EXTEND -> FAULT_HOLD [order 1] : [ArmFault]
  GRASP -> FAULT_HOLD [order 1] : [ArmFault]
  IDLE -> NAV_TO_STAGING [order 1] : after(1,sec)[MoreBoxes]
  NAV_TO_STAGING -> DOCK_SHELF [order 1] : [AtGoal && ScanDone && PerceptionValid]
  DOCK_SHELF -> ARM_EXTEND [order 1] : [AtGoal && ArmDone]
  ARM_EXTEND -> GRASP [order 2] : [ArmDone]
  IDLE -> MISSION_DONE [order 3] : after(2,sec)[~MoreBoxes && Finish && ~NeedHome]
  IDLE -> RETURN_HOME [order 2] : after(1,sec)[~MoreBoxes && NeedHome]
  FAULT_HOLD -> ARM_RETRACT [order 1] : [~ArmFault && IsTargetGrasped]
  ARM_RETRACT -> NAV_TO_TABLE [order 2] : [ArmDone]
  ARM_STOW -> RETURN_HOME : [ArmDone]
  NAV_TO_TABLE -> ARM_PLACE : [AtGoal]
  ARM_PLACE -> FAULT_HOLD [order 1] : [ArmFault]
  ARM_PLACE -> RELEASE [order 2] : [ArmDone]
  FAULT_HOLD -> ARM_STOW [order 2] : [~ArmFault && ~IsTargetGrasped]
  RELEASE -> ARM_STOW [order 1] : [~IsTargetGrasped]
  RELEASE -> ARM_STOW [order 2] : after(1,sec)
  ARM_RETRACT -> FAULT_HOLD [order 1] : [ArmFault]
  data: AtGoal input boolean; ArmDone input boolean; PerceptionValid input boolean; BoxX input double; BoxY input double; BoxZ input double; IsTargetGrasped input boolean; ArmFault input boolean; MoreBoxes input boolean; ScanDone input boolean; Finish input boolean; NeedHome input boolean; TaskState output uint8; GoalX output double; GoalY output double; IKTargetX output double; IKTargetY output double; IKTargetZ output double; GraspCmd output boolean; PlaceCmd output boolean

== matlab function WarehousePhase2Sim/Robot 1/Box Meas Pick ==
  data: pool input; y output; idx input
function y = fcn(pool,idx)
y = zeros(1,9); i = round(idx);
if i>=1 && i<=54, y(1:3) = pool(3*i-2:3*i); end

== matlab function WarehousePhase2Sim/Robot 1/Robot Pack ==
  data: c input; y output; r input; d input; c2 input
function y = fcn(c,r,d,c2)
y = [c r double(d) c2(1)];

== matlab function WarehousePhase2Sim/Robot 1/Lift Select ==
  data: q input; y output
function y = fcn(q)
y = q(1);

== matlab function WarehousePhase2Sim/Robot 1/Pose To Robot Transform ==
  data: pose input; translation output; rotation output
function [translation,rotation] = fcn(pose)
translation = [pose(1), pose(2), 0];
rotation = [pose(3), 0, 0];

== matlab function WarehousePhase2Sim/Robot 1 Cam Pose ==
  data: pose input; translation output; lift input; rotation output
function [translation,rotation] = fcn(pose,lift)
yaw=pose(3); c=cos(yaw); s=sin(yaw);
f=0.2; l=0; z=1.37+lift;
translation=[pose(1)+f*c-l*s pose(2)+f*s+l*c z];
rotation=[0 22 yaw*180/pi];

== matlab function WarehousePhase2Sim/Carton Router ==
  data: p1 input; trans output; fc input; fr input; fa input; rot output; drv output
function [trans,rot,drv] = fcn(p1,fc,fr,fa)
% every robot sends [carton(1x3) rot(1x3) drive idx]; the fleet block sends park / arrival commands. A robot that drives carton j beats the fleet.
M=54; trans=fc; rot=fr; drv=(fa>0.5);
P=[p1];
for r=1:1
  j=round(P(r,8));
  if j>=1 && j<=M && P(r,7)>0.5
    trans(3*j-2:3*j)=P(r,1:3); rot(3*j-2:3*j)=P(r,4:6); drv(j)=true;
  end
end

== matlab function WarehousePhase2Sim/Marker 1 Calc ==
  data: pose input; t1 output; r1 output; t2 output; r2 output; t3 output; r3 output
function [t1,r1,t2,r2,t3,r3] = fcn(pose)
% slat q sits at body angle (pi + th) on the chassis radius; its thin axis is radial.  Unreal frame: y negated, yaw negated.
R=0.3380; z=0.200; th=[-0.2618 0 0.2618];
p=zeros(3,3); r=zeros(3,3);
for q=1:3
  f=pose(3)+pi+th(q); p(q,:)=[pose(1)+R*cos(f) -(pose(2)+R*sin(f)) z]; r(q,:)=[0 0 -f];
end
t1=p(1,:); r1=r(1,:); t2=p(2,:); r2=r(2,:); t3=p(3,:); r3=r(3,:);

== matlab function WarehousePhase2Sim/Poses Mux ==
  data: a1 input; y output
function y = fcn(a1)
y = [reshape(a1,1,3)];

== matlab function WarehousePhase2Sim/Lifts Mux ==
  data: a1 input; y output
function y = fcn(a1)
y = [a1(1)];

== matlab function WarehousePhase2Sim/Fleet Camera Pose ==
  data: poses input; translation output; lifts input; rotation output; selPose output; selLift output; sel output
function [translation,rotation,selPose,selLift,sel] = fcn(poses,lifts)
coder.extrinsic('phase3SelRobot');
sel=1; sel=phase3SelRobot();
sel=min(max(round(sel),1),1);
selPose=poses(3*sel-2:3*sel); selLift=lifts(sel);
yaw=selPose(3); c=cos(yaw); s=sin(yaw);
f=0.2; l=0; z=1.37+selLift;
translation=[selPose(1)+f*c-l*s selPose(2)+f*s+l*c z];
rotation=[0 22 yaw*180/pi];

== matlab function WarehousePhase2Sim/Fleet Vision Viewer ==
  data: img input; ok output; pose input; lift input; sel input
function ok = fcn(img,pose,lift,sel)
coder.extrinsic('fleetVisionStep');
fleetVisionStep(img,pose,lift,sel);
ok=uint8(0);

== matlab function WarehousePhase2Sim/Robot 1/Idx Select ==
  data: c2 input; idx output
function idx = fcn(c2)
idx = c2(1);

== matlab function WarehousePhase2Sim/Pool Pack ==
  data: a1 input; y output; a2 input; a3 input; a4 input; a5 input; a6 input; a7 input; a8 input; a9 input; a10 input; a11 input; a12 input; a13 input; a14 input; a15 input; a16 input; a17 input; a18 input; a19 input; a20 input; a21 input; a22 input; a23 input; a24 input; a25 input; a26 input; a27 input; a28 input; a29 input; a30 input; a31 input; a32 input; a33 input; a34 input; a35 input; a36 input; a37 input; a38 input; a39 input; a40 input; a41 input; a42 input; a43 input; a44 input; a45 input; a46 input; a47 input; a48 input; a49 input; a50 input; a51 input; a52 input; a53 input; a54 input
function y = fcn(a1,a2,a3,a4,a5,a6,a7,a8,a9,a10,a11,a12,a13,a14,a15,a16,a17,a18,a19,a20,a21,a22,a23,a24,a25,a26,a27,a28,a29,a30,a31,a32,a33,a34,a35,a36,a37,a38,a39,a40,a41,a42,a43,a44,a45,a46,a47,a48,a49,a50,a51,a52,a53,a54)
y = [reshape(a1,1,[]) reshape(a2,1,[]) reshape(a3,1,[]) reshape(a4,1,[]) reshape(a5,1,[]) reshape(a6,1,[]) reshape(a7,1,[]) reshape(a8,1,[]) reshape(a9,1,[]) reshape(a10,1,[]) reshape(a11,1,[]) reshape(a12,1,[]) reshape(a13,1,[]) reshape(a14,1,[]) reshape(a15,1,[]) reshape(a16,1,[]) reshape(a17,1,[]) reshape(a18,1,[]) reshape(a19,1,[]) reshape(a20,1,[]) reshape(a21,1,[]) reshape(a22,1,[]) reshape(a23,1,[]) reshape(a24,1,[]) reshape(a25,1,[]) reshape(a26,1,[]) reshape(a27,1,[]) reshape(a28,1,[]) reshape(a29,1,[]) reshape(a30,1,[]) reshape(a31,1,[]) reshape(a32,1,[]) reshape(a33,1,[]) reshape(a34,1,[]) reshape(a35,1,[]) reshape(a36,1,[]) reshape(a37,1,[]) reshape(a38,1,[]) reshape(a39,1,[]) reshape(a40,1,[]) reshape(a41,1,[]) reshape(a42,1,[]) reshape(a43,1,[]) reshape(a44,1,[]) reshape(a45,1,[]) reshape(a46,1,[]) reshape(a47,1,[]) reshape(a48,1,[]) reshape(a49,1,[]) reshape(a50,1,[]) reshape(a51,1,[]) reshape(a52,1,[]) reshape(a53,1,[]) reshape(a54,1,[])];
